simulink model "A3_2_pose"  (R2024b)
settings: Solver=ode4  StartTime=0.0  StopTime=T_run  FixedStep=Ts_ctrl  RelTol=1e-3
InitFcn:
  | if ~exist('A3_model_init','file'), addpath(fileparts(get_param('A3_2_pose','FileName'))); end, A3_model_init('A3_2_pose')
StopFcn:
  | A3_model_done('A3_2_pose')
values from neighbouring files (symbols this model uses):
  alloc_mode = 2    [A3_setup.m]
  animate = 0    [A3_setup.m]
  az_prm = [half_beam; l_thr; F_max; d_max; rev_on]    [A3_setup.m]
  beta_c = deg2rad(current_direction)    [A3_setup.m]
  current_speed = 0    [A3_setup.m]
  d_rate = deg2rad(d_rate_deg)    [A3_setup.m]
  F_max = 500    [A3_azpolar_example.m]    (also in A3_nullspace_example.m; A3_pinv_example.m; A3_setup.m)
  Kb = Ki_u/Kp_u    (= 0.333333333333)    [A3_setup.m]
  Kd_psi = 200    [A3_setup.m]
  Ki_u = 100    [A3_setup.m]
  Ki_v = 100    [A3_setup.m]
  Kp_psi = 400    [A3_setup.m]
  Kp_u = 300    [A3_setup.m]
  Kp_v = 300    [A3_setup.m]
  Kp_x = 0.4    [A3_setup.m]
  Kp_y = 0.4    [A3_setup.m]
  N_max = 2*half_beam*F_max    (= 1027.135)    [A3_setup.m]
  R_stop = 1.5    [A3_setup.m]
  stop_hold = 15    [A3_setup.m]
  stop_q = [x_d; y_d; psi_d]    [A3_setup.m]
  Ts_ctrl = 0.05    [A3_setup.m]
  u_max = 1.5    [A3_setup.m]
  U_stop = 0.05    [A3_setup.m]
  usv_p = [m_usv; Izz; Xu; Xuu; Yv; Yvv; Nr; Nrr]    [A3_setup.m]
  v_max = 0.6    [A3_setup.m]
  x0 = [0.1; 0; 0; 0; 0; psi_init]    [A3_setup.m]    (also in tidy_layout.m = min(P(:,1)))
  Y_max = F_max / T_per_Y    [A3_setup.m]
libraries: slpidlib x2
settings Model: Creator=admin  LastModifiedBy=admin

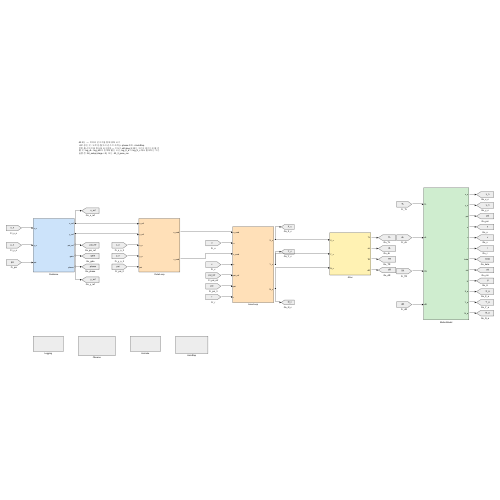
[thumbnail: Simulink's stored preview of the top-level diagram]
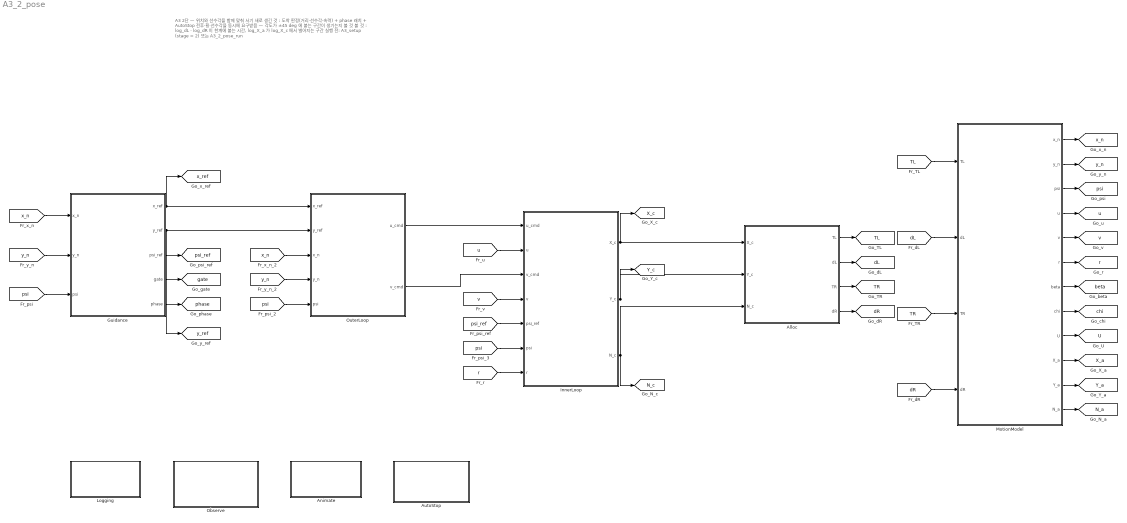
== system A3_2_pose ==
  note: A3 2단  —  위치와 선수각을 함께 맞춰 서기
      | 새로 생긴 것 : 도착 판정(거리·선수각·속력) + phase 래치 + AutoStop
      | 전후·횡·선수각을 동시에 요구받음 — 각도가 ±45 deg 에 붙는 구간이 생기는지 볼 것
      | 볼 것 : log_dL · log_dR 이 한계에 붙는 시간, log_X_a 가 log_X_c 에서 벌어지는 구간
      | 실행 전: A3_setup (stage = 2)  또는  A3_2_pose_run
  Alloc : Subsystem
  Animate : Subsystem
  AutoStop : Subsystem
  Guidance : Subsystem
  InnerLoop : Subsystem
  Logging : Subsystem
  MotionModel : Subsystem
  Observe : Subsystem
  OuterLoop : Subsystem
  tag scope: N_a=global, N_c=global, TL=global, TR=global, U=global, X_a=global, X_c=global, Y_a=global, Y_c=global, beta=global, chi=global, dL=global, dR=global, gate=global, phase=global, psi=global, psi_ref=global, r=global, u=global, v=global, x_n=global, x_ref=global, y_n=global, y_ref=global
  wires:
  InnerLoop/2(Y_c) -> Alloc/2(Y_c), [Y_c]
  OuterLoop/2(v_cmd) -> InnerLoop/3(v_cmd)
  OuterLoop/1(u_cmd) -> InnerLoop/1(u_cmd)
  Guidance/2(y_ref) -> OuterLoop/2(y_ref), [y_ref]
  Guidance/1(x_ref) -> OuterLoop/1(x_ref), [x_ref]
  InnerLoop/1(X_c) -> Alloc/1(X_c), [X_c]
  Alloc/1(TL) -> [TL]
  MotionModel/9(U) -> [U]
  MotionModel/10(X_a) -> [X_a]
  MotionModel/11(Y_a) -> [Y_a]
  MotionModel/7(beta) -> [beta]
  MotionModel/8(chi) -> [chi]
  Alloc/2(dL) -> [dL]
  Alloc/4(dR) -> [dR]
  MotionModel/3(psi) -> [psi]
  Guidance/3(psi_ref) -> [psi_ref]
  MotionModel/6(r) -> [r]
  MotionModel/4(u) -> [u]
  MotionModel/5(v) -> [v]
  MotionModel/1(x_n) -> [x_n]
  MotionModel/2(y_n) -> [y_n]
  [TL] -> MotionModel/1(TL)
  [TR] -> MotionModel/3(TR)
  [dL] -> MotionModel/2(dL)
  [dR] -> MotionModel/4(dR)
  [r] -> InnerLoop/7(r)
  [u] -> InnerLoop/2(u)
  [x_n] -> Guidance/1(x_n)
  [x_n] -> OuterLoop/3(x_n)
  [y_n] -> Guidance/2(y_n)
  [y_n] -> OuterLoop/4(y_n)
  MotionModel/12(N_a) -> [N_a]
  Alloc/3(TR) -> [TR]
  Guidance/4(gate) -> [gate]
  Guidance/5(phase) -> [phase]
  [psi] -> Guidance/3(psi)
  [psi] -> OuterLoop/5(psi)
  [psi] -> InnerLoop/6(psi)
  [psi_ref] -> InnerLoop/5(psi_ref)
  [v] -> InnerLoop/4(v)
  InnerLoop/3(N_c) -> Alloc/3(N_c), [N_c]

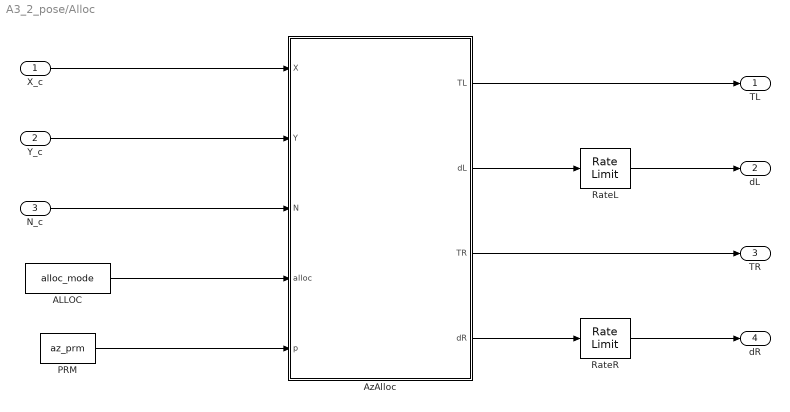
== system A3_2_pose/Alloc ==
  X_c : Inport
  Y_c : Inport  Port=2
  N_c : Inport  Port=3
  ALLOC : Constant  Value=alloc_mode
  AzAlloc : MATLAB Function  TreatAsAtomicUnit=on
  PRM : Constant  Value=az_prm
  RateL : RateLimiter  RisingSlewLimit=d_rate  FallingSlewLimit=-d_rate  SampleTimeMode=inherited
  RateR : RateLimiter  RisingSlewLimit=d_rate  FallingSlewLimit=-d_rate  SampleTimeMode=inherited
  TL : Outport
  dL : Outport  Port=2
  TR : Outport  Port=3
  dR : Outport  Port=4
  wires:
  X_c/1 -> AzAlloc/1(X)
  Y_c/1 -> AzAlloc/2(Y)
  N_c/1 -> AzAlloc/3(N)
  ALLOC/1 -> AzAlloc/4(alloc)
  PRM/1 -> AzAlloc/5(p)
  AzAlloc/2(dL) -> RateL/1
  AzAlloc/4(dR) -> RateR/1
  AzAlloc/1(TL) -> TL/1
  RateL/1 -> dL/1
  RateR/1 -> dR/1
  AzAlloc/3(TR) -> TR/1

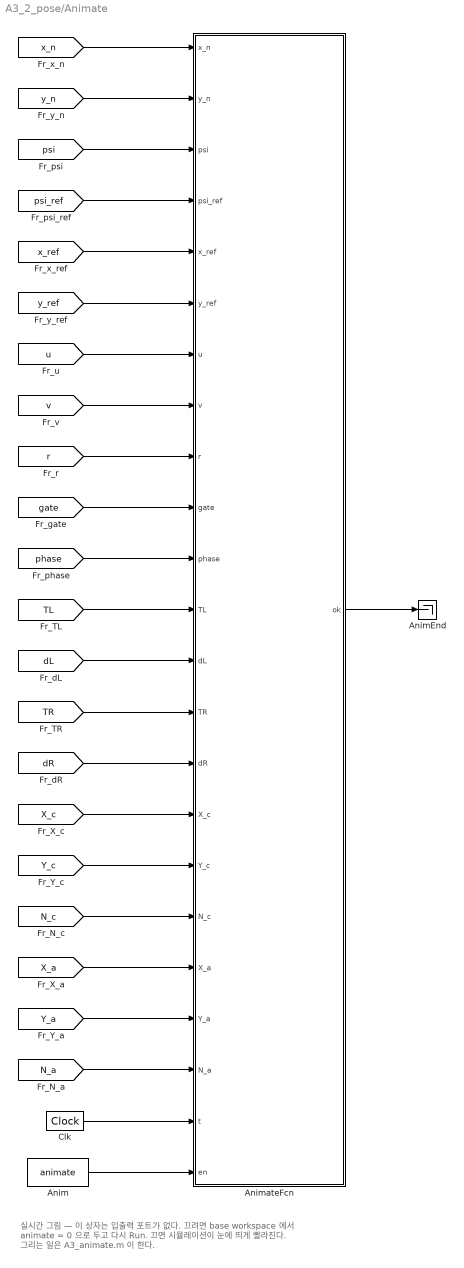
== system A3_2_pose/Animate ==
  note: 실시간 그림 — 이 상자는 입출력 포트가 없다.
      | 끄려면 base workspace 에서  animate = 0  으로 두고 다시 Run.
      | 끄면 시뮬레이션이 눈에 띄게 빨라진다.
      | 그리는 일은 A3_animate.m 이 한다.
  Anim : Constant  Value=animate
  AnimEnd : Terminator
  AnimateFcn : MATLAB Function  TreatAsAtomicUnit=on
  Clk : DigitalClock  SampleTime=Ts_ctrl
  wires:
  [x_n] -> AnimateFcn/1(x_n)
  [y_n] -> AnimateFcn/2(y_n)
  [psi] -> AnimateFcn/3(psi)
  [psi_ref] -> AnimateFcn/4(psi_ref)
  [x_ref] -> AnimateFcn/5(x_ref)
  [y_ref] -> AnimateFcn/6(y_ref)
  [u] -> AnimateFcn/7(u)
  [v] -> AnimateFcn/8(v)
  [r] -> AnimateFcn/9(r)
  [gate] -> AnimateFcn/10(gate)
  [phase] -> AnimateFcn/11(phase)
  [TL] -> AnimateFcn/12(TL)
  [dL] -> AnimateFcn/13(dL)
  [TR] -> AnimateFcn/14(TR)
  [dR] -> AnimateFcn/15(dR)
  [X_c] -> AnimateFcn/16(X_c)
  [Y_c] -> AnimateFcn/17(Y_c)
  [N_c] -> AnimateFcn/18(N_c)
  [X_a] -> AnimateFcn/19(X_a)
  [Y_a] -> AnimateFcn/20(Y_a)
  [N_a] -> AnimateFcn/21(N_a)
  Clk/1 -> AnimateFcn/22(t)
  Anim/1 -> AnimateFcn/23(en)
  AnimateFcn/1(ok) -> AnimEnd/1

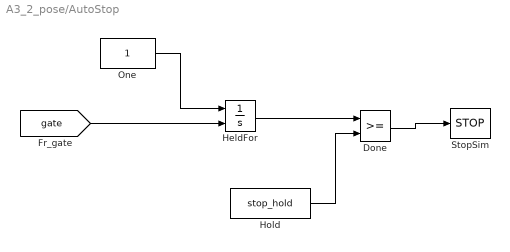
== system A3_2_pose/AutoStop ==
  Done : RelationalOperator  OutDataTypeStr=boolean  RndMeth=Simplest  InputSameDT=off
  HeldFor : Integrator  ExternalReset=level
  Hold : Constant  Value=stop_hold
  One : Constant
  StopSim : Stop
  wires:
  One/1 -> HeldFor/1
  [gate] -> HeldFor/2
  HeldFor/1 -> Done/1
  Hold/1 -> Done/2
  Done/1 -> StopSim/1

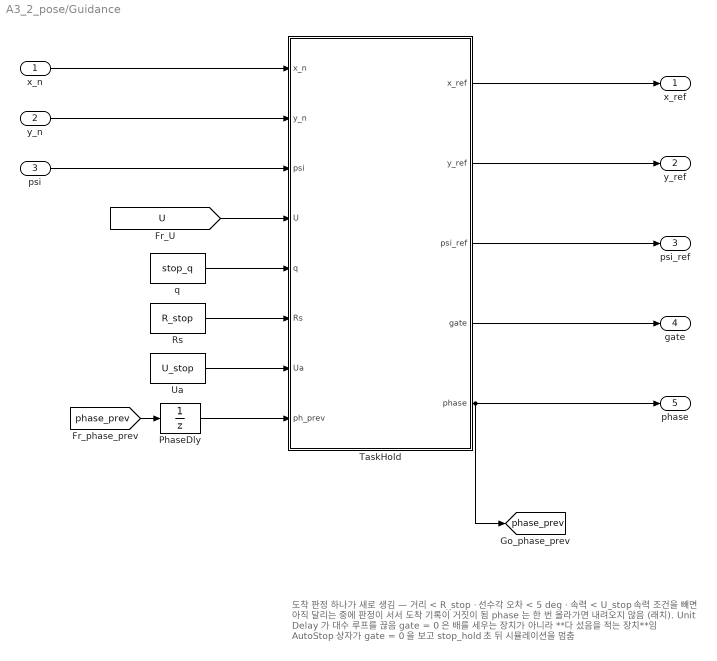
== system A3_2_pose/Guidance ==
  note: 도착 판정 하나가 새로 생김 — 거리 < R_stop · 선수각 오차 < 5 deg · 속력 < U_stop
      | 속력 조건을 빼면 아직 달리는 중에 판정이 서서 도착 기록이 거짓이 됨
      | phase 는 한 번 올라가면 내려오지 않음 (래치). Unit Delay 가 대수 루프를 끊음
      | gate = 0 은 배를 세우는 장치가 아니라 **다 섰음을 적는 장치**임
      | AutoStop 상자가 gate = 0 을 보고 stop_hold 초 뒤 시뮬레이션을 멈춤
  x_n : Inport
  y_n : Inport  Port=2
  psi : Inport  Port=3
  PhaseDly : UnitDelay  Description=phase 래치가 자기 자신을 입력으로 받으므로 그대로 되먹이면 대수 루프가 된다. 한 스텝 전 값을 쓰는 것 말고는 끊을 방법이 없는 자리다. 표본 간격을 고정 스텝(Ts_ctrl)과 같게 두어 연속 솔버(ode4)와 어긋나지 않는다.  SampleTime=Ts_ctrl  HasFrameUpgradeWarning=on
  Rs : Constant  Value=R_stop
  TaskHold : MATLAB Function  TreatAsAtomicUnit=on
  Ua : Constant  Value=U_stop
  q : Constant  Value=stop_q
  x_ref : Outport
  y_ref : Outport  Port=2
  psi_ref : Outport  Port=3
  gate : Outport  Port=4
  phase : Outport  Port=5
  tag scope: phase_prev=global
  wires:
  x_n/1 -> TaskHold/1(x_n)
  y_n/1 -> TaskHold/2(y_n)
  psi/1 -> TaskHold/3(psi)
  [U] -> TaskHold/4(U)
  q/1 -> TaskHold/5(q)
  Rs/1 -> TaskHold/6(Rs)
  Ua/1 -> TaskHold/7(Ua)
  PhaseDly/1 -> TaskHold/8(ph_prev)
  TaskHold/1(x_ref) -> x_ref/1
  TaskHold/2(y_ref) -> y_ref/1
  TaskHold/3(psi_ref) -> psi_ref/1
  TaskHold/4(gate) -> gate/1
  TaskHold/5(phase) -> phase/1, [phase_prev]
  [phase_prev] -> PhaseDly/1

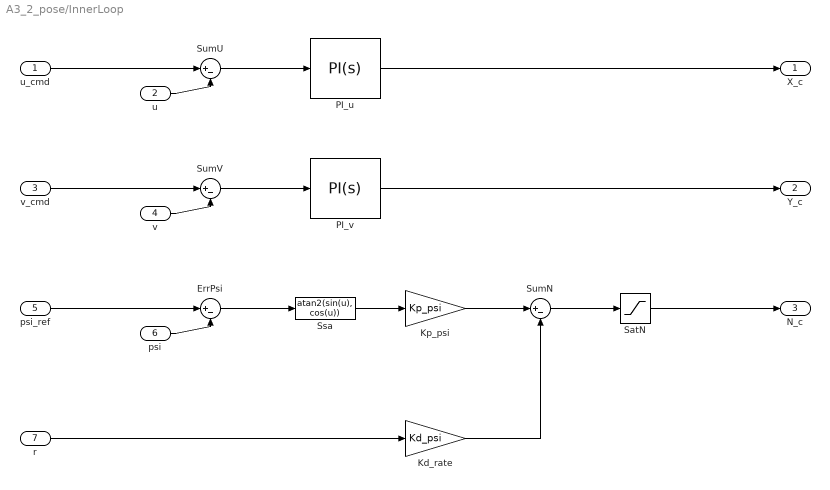
== system A3_2_pose/InnerLoop ==
  u_cmd : Inport
  u : Inport  Port=2
  v_cmd : Inport  Port=3
  v : Inport  Port=4
  psi_ref : Inport  Port=5
  psi : Inport  Port=6
  r : Inport  Port=7
  ErrPsi : Sum  Inputs=|+-
  Kd_rate : Gain  Gain=Kd_psi
  Kp_psi : Gain  Gain=Kp_psi
  PI_u : slpidlib/PID Controller  Controller=PI  Form=Parallel  TimeDomain=Continuous-time  UseExternalTs=off  SampleTime=-1  IntegratorMethod=Forward Euler  FilterMethod=Forward Euler  ControllerParametersSource=internal  P=Kp_u  I=Ki_u  UseKiTs=off  D=0  UseExternalDerivativeSource=off  N=100  UseFilter=on  TunerSelectOption=Transfer Function Based (PID Tuner App)  InitialConditionSource=internal  InitialConditionForIntegrator=0  InitialConditionForFilter=0  DifferentiatorICPrevScaledInput=0  ExternalReset=none  TrackingMode=off  Kt=1  LimitOutput=on  SatLimitsSource=internal  UpperSaturationLimit=2*F_max  LowerSaturationLimit=-(2*F_max)  LinearizeAsGain=on  AntiWindupMode=back-calculation  Kb=Kb  LimitIntegrator=off  UpperIntegratorSaturationLimit=inf  LowerIntegratorSaturationLimit=-inf  POutMin=[]  POutMax=[]  IOutMin=[]  IOutMax=[]  DOutMin=[]  DOutMax=[]  NOutMin=[]  NOutMax=[]  SumOutMin=[]  SumOutMax=[]  SaturationOutMin=[]  SaturationOutMax=[]  PParamMin=[]  PParamMax=[]  IParamMin=[]  IParamMax=[]  DParamMin=[]  DParamMax=[]  NParamMin=[]  NParamMax=[]  KbParamMin=[]  KbParamMax=[]  KtParamMin=[]  KtParamMax=[]  KbOutMin=[]  KbOutMax=[]  KtOutMin=[]  KtOutMax=[]  IntegratorOutMin=[]  IntegratorOutMax=[]  FilterOutMin=[]  FilterOutMax=[]  SumI1OutMin=[]  SumI1OutMax=[]  SumI2OutMin=[]  SumI2OutMax=[]  SumI3OutMin=[]  SumI3OutMax=[]  SumI4OutMin=[]  SumI4OutMax=[]  SumDOutMin=[]  SumDOutMax=[]  DifferentiatorOutMin=[]  DifferentiatorOutMax=[]  FilterDiffOutCoefMin=[]  FilterDiffOutCoefMax=[]  ReciprocalOutMin=[]  ReciprocalOutMax=[]  SumDenOutMin=[]  SumDenOutMax=[]  SumNumOutMin=[]  SumNumOutMax=[]  DivideOutMin=[]  DivideOutMax=[]  UdiffTsProdOutMin=[]  UdiffTsProdOutMax=[]  NTsProdOutMin=[]  NTsProdOutMax=[]  UintegralTsProdOutMin=[]  UintegralTsProdOutMax=[]  UngainTsProdOutMin=[]  UngainTsProdOutMax=[]  ClampingZeroOutDataTypeStr=Inherit: Inherit via back propagation  ClampingZeroOutMin=[]  ClampingZeroOutMax=[]  FilterDenConstantOutDataTypeStr=Inherit: Inherit via back propagation  FilterDenConstantOutMin=[]  FilterDenConstantOutMax=[]  PCopyOutDataTypeStr=Inherit: Inherit via back propagation  PCopyOutMin=[]  PCopyOutMax=[]  NCopyOutDataTypeStr=Inherit: Inherit via back propagation  NCopyOutMin=[]  NCopyOutMax=[]  IntegratorContinuousStateAttributes=''  IntegratorStateMustResolveToSignalObject=off  IntegratorRTWStateStorageClass=Auto  FilterContinuousStateAttributes=''  FilterStateMustResolveToSignalObject=off  FilterRTWStateStorageClass=Auto  ParallelPVariant=InternalParameters  IdealPVariant=Disabled  IVariant=InternalParameters  DVariant=Disabled  IntegratorVariant=Continuous  SatVariant=Enabled  AWVariant=BackCalculation  PCopyVariant=Disabled  TRVariant=Disabled  FdbkBlocksVariant=Forward  IdealPFdbkVariant=Disabled  SatFdbkVariant=Disabled  DerivativeFilterVariant=Disabled  NVariant=Disabled  NCopyVariant=Disabled_SignalSpec  FilterICVariant=Disabled  IntegratorICVariant=InternalICs  ExternalResetVariant=Disabled  TRSumVariant=Passthrough  SumFdbkVariant=Disabled  SumVariant=Sum_PI  TsampFilterVariant=InternalTs  TsampNgainVariant=Passthrough  TsampIntegralVariant=Disabled_SignalSpec  ExternalSaturationOutDataTypeStr=Inherit: Same as second input  DerivativeSourceVariant=Disabled  PreIntVariant=InternalPreInt
  PI_v : slpidlib/PID Controller  Controller=PI  Form=Parallel  TimeDomain=Continuous-time  UseExternalTs=off  SampleTime=-1  IntegratorMethod=Forward Euler  FilterMethod=Forward Euler  ControllerParametersSource=internal  P=Kp_v  I=Ki_v  UseKiTs=off  D=0  UseExternalDerivativeSource=off  N=100  UseFilter=on  TunerSelectOption=Transfer Function Based (PID Tuner App)  InitialConditionSource=internal  InitialConditionForIntegrator=0  InitialConditionForFilter=0  DifferentiatorICPrevScaledInput=0  ExternalReset=none  TrackingMode=off  Kt=1  LimitOutput=on  SatLimitsSource=internal  UpperSaturationLimit=Y_max  LowerSaturationLimit=-(Y_max)  LinearizeAsGain=on  AntiWindupMode=back-calculation  Kb=Kb  LimitIntegrator=off  UpperIntegratorSaturationLimit=inf  LowerIntegratorSaturationLimit=-inf  POutMin=[]  POutMax=[]  IOutMin=[]  IOutMax=[]  DOutMin=[]  DOutMax=[]  NOutMin=[]  NOutMax=[]  SumOutMin=[]  SumOutMax=[]  SaturationOutMin=[]  SaturationOutMax=[]  PParamMin=[]  PParamMax=[]  IParamMin=[]  IParamMax=[]  DParamMin=[]  DParamMax=[]  NParamMin=[]  NParamMax=[]  KbParamMin=[]  KbParamMax=[]  KtParamMin=[]  KtParamMax=[]  KbOutMin=[]  KbOutMax=[]  KtOutMin=[]  KtOutMax=[]  IntegratorOutMin=[]  IntegratorOutMax=[]  FilterOutMin=[]  FilterOutMax=[]  SumI1OutMin=[]  SumI1OutMax=[]  SumI2OutMin=[]  SumI2OutMax=[]  SumI3OutMin=[]  SumI3OutMax=[]  SumI4OutMin=[]  SumI4OutMax=[]  SumDOutMin=[]  SumDOutMax=[]  DifferentiatorOutMin=[]  DifferentiatorOutMax=[]  FilterDiffOutCoefMin=[]  FilterDiffOutCoefMax=[]  ReciprocalOutMin=[]  ReciprocalOutMax=[]  SumDenOutMin=[]  SumDenOutMax=[]  SumNumOutMin=[]  SumNumOutMax=[]  DivideOutMin=[]  DivideOutMax=[]  UdiffTsProdOutMin=[]  UdiffTsProdOutMax=[]  NTsProdOutMin=[]  NTsProdOutMax=[]  UintegralTsProdOutMin=[]  UintegralTsProdOutMax=[]  UngainTsProdOutMin=[]  UngainTsProdOutMax=[]  ClampingZeroOutDataTypeStr=Inherit: Inherit via back propagation  ClampingZeroOutMin=[]  ClampingZeroOutMax=[]  FilterDenConstantOutDataTypeStr=Inherit: Inherit via back propagation  FilterDenConstantOutMin=[]  FilterDenConstantOutMax=[]  PCopyOutDataTypeStr=Inherit: Inherit via back propagation  PCopyOutMin=[]  PCopyOutMax=[]  NCopyOutDataTypeStr=Inherit: Inherit via back propagation  NCopyOutMin=[]  NCopyOutMax=[]  IntegratorContinuousStateAttributes=''  IntegratorStateMustResolveToSignalObject=off  IntegratorRTWStateStorageClass=Auto  FilterContinuousStateAttributes=''  FilterStateMustResolveToSignalObject=off  FilterRTWStateStorageClass=Auto  ParallelPVariant=InternalParameters  IdealPVariant=Disabled  IVariant=InternalParameters  DVariant=Disabled  IntegratorVariant=Continuous  SatVariant=Enabled  AWVariant=BackCalculation  PCopyVariant=Disabled  TRVariant=Disabled  FdbkBlocksVariant=Forward  IdealPFdbkVariant=Disabled  SatFdbkVariant=Disabled  DerivativeFilterVariant=Disabled  NVariant=Disabled  NCopyVariant=Disabled_SignalSpec  FilterICVariant=Disabled  IntegratorICVariant=InternalICs  ExternalResetVariant=Disabled  TRSumVariant=Passthrough  SumFdbkVariant=Disabled  SumVariant=Sum_PI  TsampFilterVariant=InternalTs  TsampNgainVariant=Passthrough  TsampIntegralVariant=Disabled_SignalSpec  ExternalSaturationOutDataTypeStr=Inherit: Same as second input  DerivativeSourceVariant=Disabled  PreIntVariant=InternalPreInt
  SatN : Saturate  UpperLimit=N_max  LowerLimit=-(N_max)
  Ssa : Fcn  Expr=atan2(sin(u), cos(u))
  SumN : Sum  Inputs=|+-
  SumU : Sum  Inputs=|+-
  SumV : Sum  Inputs=|+-
  X_c : Outport
  Y_c : Outport  Port=2
  N_c : Outport  Port=3
  wires:
  u_cmd/1 -> SumU/1
  u/1 -> SumU/2
  v_cmd/1 -> SumV/1
  v/1 -> SumV/2
  SumU/1 -> PI_u/1
  SumV/1 -> PI_v/1
  ErrPsi/1 -> Ssa/1
  psi_ref/1 -> ErrPsi/1
  psi/1 -> ErrPsi/2
  Ssa/1 -> Kp_psi/1
  r/1 -> Kd_rate/1
  Kp_psi/1 -> SumN/1
  Kd_rate/1 -> SumN/2
  SumN/1 -> SatN/1
  PI_u/1 -> X_c/1
  SatN/1 -> N_c/1
  PI_v/1 -> Y_c/1

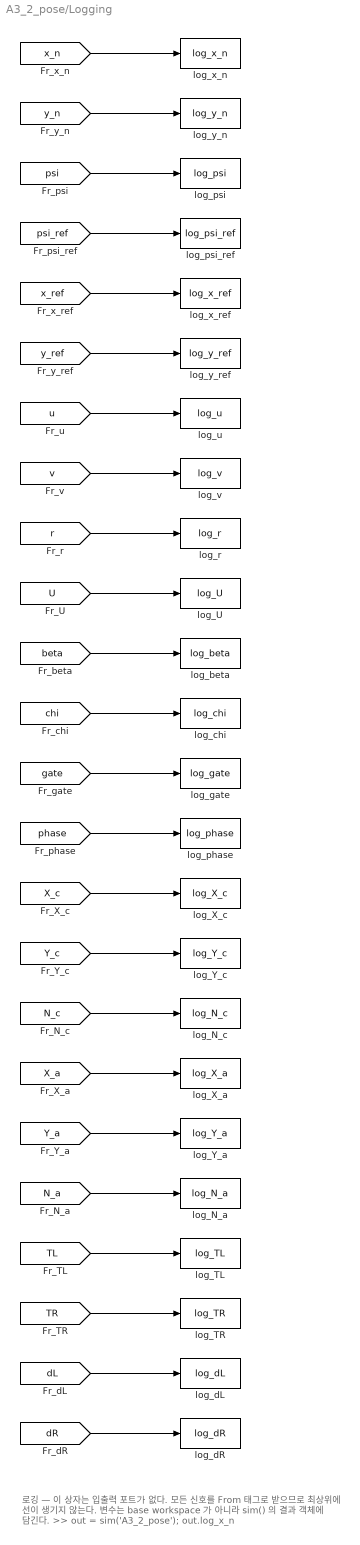
== system A3_2_pose/Logging ==
  note: 로깅 — 이 상자는 입출력 포트가 없다.
      | 모든 신호를 From 태그로 받으므로 최상위에 선이 생기지 않는다.
      | 변수는 base workspace 가 아니라 sim() 의 결과 객체에 담긴다.
      |   >> out = sim('A3_2_pose');  out.log_x_n
  log_N_a : ToWorkspace  VariableName=log_N_a  SaveFormat=Timeseries  SampleTime=Ts_ctrl
  log_N_c : ToWorkspace  VariableName=log_N_c  SaveFormat=Timeseries  SampleTime=Ts_ctrl
  log_TL : ToWorkspace  VariableName=log_TL  SaveFormat=Timeseries  SampleTime=Ts_ctrl
  log_TR : ToWorkspace  VariableName=log_TR  SaveFormat=Timeseries  SampleTime=Ts_ctrl
  log_U : ToWorkspace  VariableName=log_U  SaveFormat=Timeseries  SampleTime=Ts_ctrl
  log_X_a : ToWorkspace  VariableName=log_X_a  SaveFormat=Timeseries  SampleTime=Ts_ctrl
  log_X_c : ToWorkspace  VariableName=log_X_c  SaveFormat=Timeseries  SampleTime=Ts_ctrl
  log_Y_a : ToWorkspace  VariableName=log_Y_a  SaveFormat=Timeseries  SampleTime=Ts_ctrl
  log_Y_c : ToWorkspace  VariableName=log_Y_c  SaveFormat=Timeseries  SampleTime=Ts_ctrl
  log_beta : ToWorkspace  VariableName=log_beta  SaveFormat=Timeseries  SampleTime=Ts_ctrl
  log_chi : ToWorkspace  VariableName=log_chi  SaveFormat=Timeseries  SampleTime=Ts_ctrl
  log_dL : ToWorkspace  VariableName=log_dL  SaveFormat=Timeseries  SampleTime=Ts_ctrl
  log_dR : ToWorkspace  VariableName=log_dR  SaveFormat=Timeseries  SampleTime=Ts_ctrl
  log_gate : ToWorkspace  VariableName=log_gate  SaveFormat=Timeseries  SampleTime=Ts_ctrl
  log_phase : ToWorkspace  VariableName=log_phase  SaveFormat=Timeseries  SampleTime=Ts_ctrl
  log_psi : ToWorkspace  VariableName=log_psi  SaveFormat=Timeseries  SampleTime=Ts_ctrl
  log_psi_ref : ToWorkspace  VariableName=log_psi_ref  SaveFormat=Timeseries  SampleTime=Ts_ctrl
  log_r : ToWorkspace  VariableName=log_r  SaveFormat=Timeseries  SampleTime=Ts_ctrl
  log_u : ToWorkspace  VariableName=log_u  SaveFormat=Timeseries  SampleTime=Ts_ctrl
  log_v : ToWorkspace  VariableName=log_v  SaveFormat=Timeseries  SampleTime=Ts_ctrl
  log_x_n : ToWorkspace  VariableName=log_x_n  SaveFormat=Timeseries  SampleTime=Ts_ctrl
  log_x_ref : ToWorkspace  VariableName=log_x_ref  SaveFormat=Timeseries  SampleTime=Ts_ctrl
  log_y_n : ToWorkspace  VariableName=log_y_n  SaveFormat=Timeseries  SampleTime=Ts_ctrl
  log_y_ref : ToWorkspace  VariableName=log_y_ref  SaveFormat=Timeseries  SampleTime=Ts_ctrl
  wires:
  [x_n] -> log_x_n/1
  [y_n] -> log_y_n/1
  [psi] -> log_psi/1
  [psi_ref] -> log_psi_ref/1
  [x_ref] -> log_x_ref/1
  [y_ref] -> log_y_ref/1
  [u] -> log_u/1
  [v] -> log_v/1
  [r] -> log_r/1
  [U] -> log_U/1
  [beta] -> log_beta/1
  [chi] -> log_chi/1
  [gate] -> log_gate/1
  [phase] -> log_phase/1
  [X_c] -> log_X_c/1
  [Y_c] -> log_Y_c/1
  [N_c] -> log_N_c/1
  [X_a] -> log_X_a/1
  [Y_a] -> log_Y_a/1
  [N_a] -> log_N_a/1
  [TL] -> log_TL/1
  [TR] -> log_TR/1
  [dL] -> log_dL/1
  [dR] -> log_dR/1

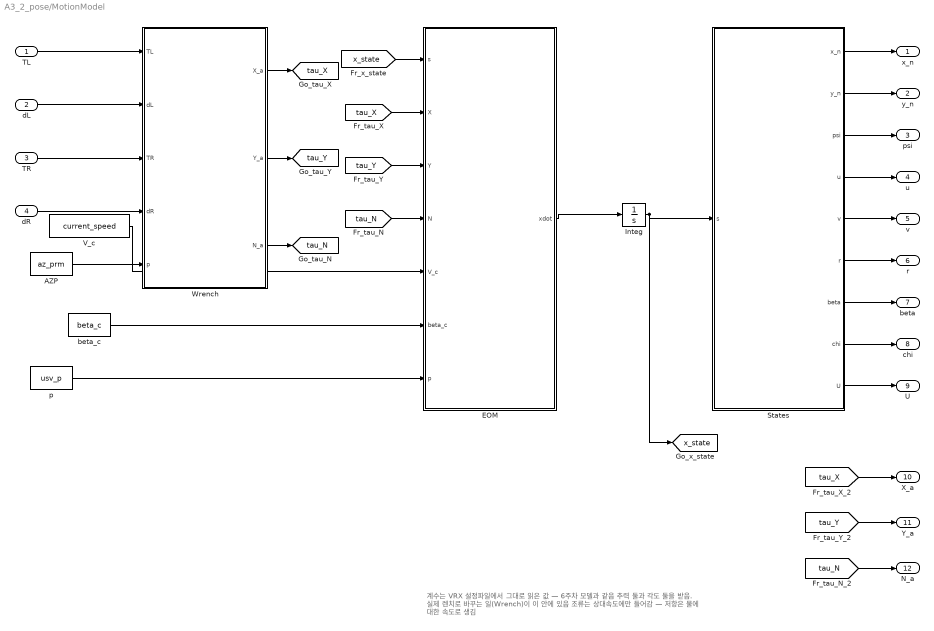
== system A3_2_pose/MotionModel ==
  note: 계수는 VRX 설정파일에서 그대로 읽은 값 — 6주차 모델과 같음
      | 추력 둘과 각도 둘을 받음. 실제 렌치로 바꾸는 일(Wrench)이 이 안에 있음
      | 조류는 상대속도에만 들어감 — 저항은 물에 대한 속도로 생김
  TL : Inport
  dL : Inport  Port=2
  TR : Inport  Port=3
  dR : Inport  Port=4
  AZP : Constant  Value=az_prm
  EOM : MATLAB Function  TreatAsAtomicUnit=on
  Integ : Integrator  InitialCondition=x0
  States : MATLAB Function  TreatAsAtomicUnit=on
  V_c : Constant  Value=current_speed
  Wrench : MATLAB Function  TreatAsAtomicUnit=on
  beta_c : Constant  Value=beta_c
  p : Constant  Value=usv_p
  x_n : Outport
  y_n : Outport  Port=2
  psi : Outport  Port=3
  u : Outport  Port=4
  v : Outport  Port=5
  r : Outport  Port=6
  beta : Outport  Port=7
  chi : Outport  Port=8
  U : Outport  Port=9
  X_a : Outport  Port=10
  Y_a : Outport  Port=11
  N_a : Outport  Port=12
  tag scope: tau_N=global, tau_X=global, tau_Y=global, x_state=global
  wires:
  TL/1 -> Wrench/1(TL)
  dL/1 -> Wrench/2(dL)
  TR/1 -> Wrench/3(TR)
  dR/1 -> Wrench/4(dR)
  AZP/1 -> Wrench/5(p)
  Wrench/1(X_a) -> [tau_X]
  Wrench/2(Y_a) -> [tau_Y]
  Wrench/3(N_a) -> [tau_N]
  [tau_X] -> EOM/2(X)
  [tau_Y] -> EOM/3(Y)
  [tau_N] -> EOM/4(N)
  V_c/1 -> EOM/5(V_c)
  beta_c/1 -> EOM/6(beta_c)
  p/1 -> EOM/7(p)
  EOM/1(xdot) -> Integ/1
  Integ/1 -> States/1(s), [x_state]
  [x_state] -> EOM/1(s)
  States/1(x_n) -> x_n/1
  States/2(y_n) -> y_n/1
  States/3(psi) -> psi/1
  States/4(u) -> u/1
  States/5(v) -> v/1
  States/6(r) -> r/1
  States/7(beta) -> beta/1
  States/8(chi) -> chi/1
  States/9(U) -> U/1
  [tau_X] -> X_a/1
  [tau_Y] -> Y_a/1
  [tau_N] -> N_a/1

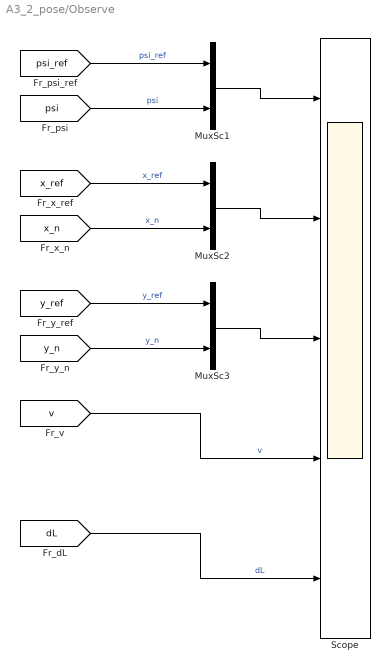
== system A3_2_pose/Observe ==
  MuxSc1 : Mux  Inputs=2
  MuxSc2 : Mux  Inputs=2
  MuxSc3 : Mux  Inputs=2
  Scope : Scope  NumInputPorts=5
  wires:
  [psi_ref] -> MuxSc1/1  "psi_ref"
  [psi] -> MuxSc1/2  "psi"
  MuxSc1/1 -> Scope/1
  [x_ref] -> MuxSc2/1  "x_ref"
  [x_n] -> MuxSc2/2  "x_n"
  MuxSc2/1 -> Scope/2
  [y_ref] -> MuxSc3/1  "y_ref"
  [y_n] -> MuxSc3/2  "y_n"
  MuxSc3/1 -> Scope/3
  [v] -> Scope/4  "v"
  [dL] -> Scope/5  "dL"

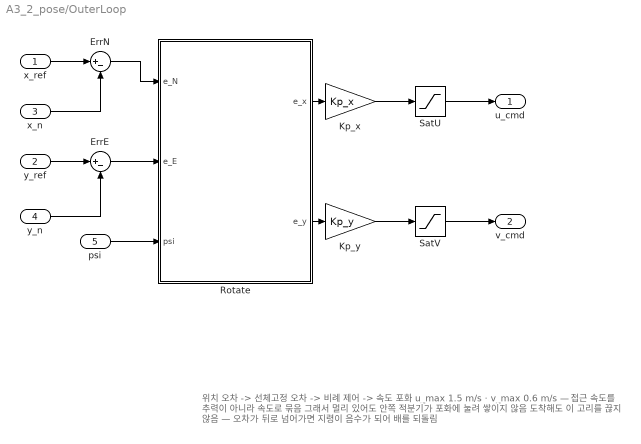
== system A3_2_pose/OuterLoop ==
  note: 위치 오차 -> 선체고정 오차 -> 비례 제어 -> 속도 포화
      | u_max 1.5 m/s · v_max 0.6 m/s — 접근 속도를 추력이 아니라 속도로 묶음
      | 그래서 멀리 있어도 안쪽 적분기가 포화에 눌려 쌓이지 않음
      | 도착해도 이 고리를 끊지 않음 — 오차가 뒤로 넘어가면 지령이 음수가 되어 배를 되돌림
  x_ref : Inport
  y_ref : Inport  Port=2
  x_n : Inport  Port=3
  y_n : Inport  Port=4
  psi : Inport  Port=5
  ErrE : Sum  Inputs=|+-
  ErrN : Sum  Inputs=|+-
  Kp_x : Gain  Gain=Kp_x
  Kp_y : Gain  Gain=Kp_y
  Rotate : MATLAB Function  TreatAsAtomicUnit=on
  SatU : Saturate  UpperLimit=u_max  LowerLimit=-(u_max)
  SatV : Saturate  UpperLimit=v_max  LowerLimit=-(v_max)
  u_cmd : Outport
  v_cmd : Outport  Port=2
  wires:
  x_ref/1 -> ErrN/1
  Rotate/1(e_x) -> Kp_x/1
  Rotate/2(e_y) -> Kp_y/1
  ErrE/1 -> Rotate/2(e_E)
  x_n/1 -> ErrN/2
  y_ref/1 -> ErrE/1
  ErrN/1 -> Rotate/1(e_N)
  y_n/1 -> ErrE/2
  psi/1 -> Rotate/3(psi)
  Kp_x/1 -> SatU/1
  Kp_y/1 -> SatV/1
  SatU/1 -> u_cmd/1
  SatV/1 -> v_cmd/1

== matlab function A3_2_pose/Animate/AnimateFcn ==
  data: x_n input; y_n input; psi input; psi_ref input; x_ref input; y_ref input; u input; ok output; v input; r input; gate input; phase input; TL input; dL input; TR input; dR input; X_c input; Y_c input; N_c input; X_a input; Y_a input; N_a input; t input; en input
function ok = AnimateFcn(x_n, y_n, psi, psi_ref, x_ref, y_ref, u, v, r, gate, phase, TL, dL, TR, dR, X_c, Y_c, N_c, X_a, Y_a, N_a, t, en)
%#codegen
% Live plot while the model runs. A MATLAB Function block cannot
% plot, so the drawing function is declared extrinsic: Simulink
% calls plain MATLAB instead of generating code for it.
coder.extrinsic('A3_animate');
ok = 1;
if en > 0.5
    A3_animate(x_n, y_n, psi, psi_ref, x_ref, y_ref, u, v, r, gate, phase, TL, dL, TR, dR, X_c, Y_c, N_c, X_a, Y_a, N_a, t);
end

== matlab function A3_2_pose/OuterLoop/Rotate ==
  data: e_N input; e_x output; e_E input; psi input; e_y output
function [e_x, e_y] = Rotate(e_N, e_E, psi)
%#codegen
%  NED 위치 오차를 선체고정 오차로 돌린다. e_x 앞쪽, e_y 우현쪽 [m]
e_x =  cos(psi)*e_N + sin(psi)*e_E;
e_y = -sin(psi)*e_N + cos(psi)*e_E;

== matlab function A3_2_pose/Guidance/TaskHold ==
  data: x_n input; x_ref output; y_n input; psi input; U input; q input; Rs input; Ua input; ph_prev input; y_ref output; psi_ref output; gate output; phase output
function [x_ref, y_ref, psi_ref, gate, phase] = TaskHold(x_n, y_n, psi, U, q, Rs, Ua, ph_prev)
%#codegen
%  한 점·한 선수각을 목표로 주고, 거기 가서 **섰는지** 판정한다.
%
%    U  = 대지속력 [m/s]      운동모델이 낸 sqrt(u^2 + v^2)
%    q  = [x_d; y_d; psi_d]   목표 자세 (psi_d 는 rad)
%    Rs = R_stop              도착으로 보는 반지름 [m]
%    Ua = U_stop              도착으로 보는 속력 한계 [m/s]
%
%  gate = 1 이면 바깥 고리가 속도 지령을 낸다. 0 이면 0 을 내어 배가 선다.
x_ref = q(1);  y_ref = q(2);  psi_ref = q(3);
d = sqrt((x_ref - x_n)^2 + (y_ref - y_n)^2);
e = atan2(sin(psi_ref - psi), cos(psi_ref - psi));
ph = ph_prev;
if ph < 1 && d < Rs && abs(e) < 5*pi/180 && U < Ua
    ph = 1;                   %  도착 — 한 번 올라가면 내려오지 않는다
end
phase = ph;
gate  = double(ph < 1);

== matlab function A3_2_pose/Alloc/AzAlloc ==
  data: X input; TL output; Y input; N input; alloc input; p input; dL output; TR output; dR output
function [TL, dL, TR, dR] = AzAlloc(X, Y, N, alloc, p)
%#codegen
%  아지무스 추진기 둘에 요구 렌치를 나누어 준다
%
%  == 입력 ==============================================================
%    X      요구 전후 힘   [N]      선수 방향(+앞)
%    Y      요구 횡 힘     [N]      우현 방향(+오른쪽)
%    N      요구 요 모멘트 [N m]    시계 방향(+우선회)
%    alloc  배분 방식 [-]           1 = pseudo-inverse
%                                   2 = pseudo-inverse + null space 보정
%    p      기하·한계 묶음 (A3_setup.m 의 az_prm)
%      p(1) = b     반폭        [m]    중심선에서 추진기까지
%      p(2) = L     거리        [m]    무게중심에서 추진기까지 (뒤쪽)
%      p(3) = Fmax  추력 한계   [N]    한 대 기준
%      p(4) = dmax  각도 한계   [rad]
%      p(5) = rev   추력 반전   [-]    1 = 허용, 0 = 금지
%
%  == 출력 ==============================================================
%    TL, TR   좌·우 추력   [N]    양수면 노즐이 보는 쪽으로 민다
%    dL, dR   좌·우 각도   [rad]  선수 기준, 우현 쪽이 +
%
%  == 왜 추력과 각도를 바로 풀지 않는가 ================================
%    추진기 한 대의 힘은 극좌표 (T, d) 로 쓰면 비선형이다
%        Fx = T cos(d),   Fy = T sin(d)
%    그래서 추력과 각도를 묶어 **직교 성분 넷**을 미지수로 둔다
%        ue = [Fx_L; Fy_L; Fx_R; Fy_R]        (확장 추력 벡터)
%    이렇게 두면 요구 렌치와의 관계가 **완전한 선형식**이 된다
%        B ue = tau,   tau = [X; Y; N]
%    B 의 각 열은 "그 성분 1 N 이 렌치에 얼마를 보태는가" 이다
%    풀고 난 뒤에 극좌표로 되돌리면 추력과 각도가 나온다 (3 단계)
%    이 방식은 Sarda 등 [1] 6 절이 실제 WAM-V 에 쓴 것과 같다
%
%  == 해가 하나가 아니다 ================================================
%    미지수 4 개, 식 3 개 — 같은 렌치를 내는 해가 **직선 하나**를 이룬다
%      alloc = 1   그 직선에서 원점에 가장 가까운 점 (pseudo-inverse)
%      alloc = 2   각도 한계를 지키는 점으로 직선 위를 미끄러진다
%    직선의 방향 n = [0; 1; 0; -1] 은 좌우 횡력만 주고받는 꼴이라
%    얼마를 더해도 X, Y, N 이 한 톨도 변하지 않는다 (B n = 0)
%
%  == 참고 문헌 ==========================================================
%    [1] Sarda, Qu, Bertaska, von Ellenrieder (2016)
%        "Station keeping control of an unmanned surface vehicle exposed
%         to current and wind disturbances", Ocean Engineering 127, 305-324
%        6 절 — 아지무스 WAM-V 의 확장 추력 벡터와 pseudo-inverse 배분
%    [2] Sordalen (1997) "Optimal thrust allocation for marine vessels",
%        Control Engineering Practice 5(9), 1223-1231 — null space 이용
%    [3] Fossen (2021) "Handbook of Marine Craft Hydrodynamics and Motion
%        Control", 2nd ed., 11 장 — 배분 행렬과 pseudo-inverse 일반론

b = p(1);  L = p(2);  Fmax = p(3);  dmax = p(4);  rev = p(5);

tau = [X; Y; N];

%  배분 행렬 — 열 하나가 성분 하나의 몫이다
%    1 행 전후 · 2 행 횡 · 3 행 요 모멘트
%    좌현은 (x, y) = (-L, -b), 우현은 (-L, +b) 에 앉는다
B = [ 1,  0,  1,  0; ...
      0,  1,  0,  1; ...
      b, -L, -b, -L];

%  === 1 단계. pseudo-inverse — 크기가 가장 작은 해 ===================
%    ue = B' (B B')^-1 tau.  해의 직선에서 원점에 가장 가까운 점이다
ue = B' * ((B*B') \ tau);

%  === 2 단계. null space 보정 (alloc = 2) ============================
%    각도 한계는 |Fy| <= tan(dmax) |Fx| 와 같은 말이다.
%    ue + lam*n 을 넣으면 lam 에 대해 1 차식이라 허용 구간이 바로 나온다
if alloc > 1.5
    nz = [0; 1; 0; -1];
    td = tan(dmax);
    lo = max(-td*abs(ue(1)) - ue(2),  ue(4) - td*abs(ue(3)));
    hi = min( td*abs(ue(1)) - ue(2),  ue(4) + td*abs(ue(3)));
    if lo <= hi
        lam = min(max(0, lo), hi);     % 구간 안에서 0 에 가장 가까운 값
    else
        lam = (lo + hi)/2;             % 구간이 비면 가운데 — 덜 넘긴다
    end
    ue = ue + lam*nz;
end

%  === 3 단계. 극좌표로 되돌리고 한계 안으로 넣는다 ===================
[TL, dL] = az_polar(ue(1), ue(2), Fmax, dmax, rev);
[TR, dR] = az_polar(ue(3), ue(4), Fmax, dmax, rev);


function [T, d] = az_polar(Fx, Fy, Fmax, dmax, rev)
%  직교 성분 둘 -> 추력 하나와 각도 하나
T = hypot(Fx, Fy);
d = atan2(Fy, Fx);

%  뒤쪽을 보라는 요구는 **앞을 보고 역추력** 으로 바꿔 쓴다 (같은 힘)
if abs(d) > pi/2
    d = d - sign(d)*pi;
    T = -T;
end

%  역추력을 금지했으면 되돌린다 — 각도가 한계를 넘게 된다 (A3-4 실습)
if rev < 0.5 && T < 0
    T = -T;
    d = d + sign(d + (d==0))*pi;
    if d >  pi, d = d - 2*pi; end
    if d < -pi, d = d + 2*pi; end
end

%  한계 — 각도와 추력을 각각 한 줄로 깎는다
%    깎인 만큼이 "못 낸 힘" 으로 남아 운동모델 쪽 기록에 숫자로 보인다
d = max(min(d,  dmax), -dmax);
T = max(min(T,  Fmax), -Fmax);

== matlab function A3_2_pose/MotionModel/Wrench ==
  data: TL input; X_a output; dL input; TR input; dR input; p input; Y_a output; N_a output
function [X_a, Y_a, N_a] = Wrench(TL, dL, TR, dR, p)
%#codegen
%  추진기 명령 -> 선체에 걸리는 렌치 (운동모델의 입구)
%
%  == 입력 ==============================================================
%    TL, TR   좌·우 추력 [N]      배분기가 낸 값. 음수면 역추력
%    dL, dR   좌·우 각도 [rad]    변화율 제한을 거친 실제 각도
%    p        기하 묶음 — p(1) = b 반폭 [m], p(2) = L 거리 [m]
%
%  == 출력 ==============================================================
%    X_a  실제 전후 힘   [N]
%    Y_a  실제 횡 힘     [N]
%    N_a  실제 요 모멘트 [N m]
%
%  == 왜 운동모델 안에 있는가 ===========================================
%    선체가 받는 것은 추력과 각도가 아니라 **힘과 모멘트**다. 추진기가
%    어떻게 달려 있는지가 그 변환을 정하므로, 변환은 배(운동모델) 쪽에
%    속한다. 배분기는 "무엇을 명령할까" 까지만 책임진다
%
%  == 배분기와 같은 행렬이다 ============================================
%    배분기는 B ue = tau 를 **거꾸로** 풀었고, 여기서는 **바로** 쓴다
%        ue = [TL cos(dL); TL sin(dL); TR cos(dR); TR sin(dR)]
%        tau_a = B ue
%    각도·추력 한계에 물리지 않으면 tau_a 가 요구 렌치와 같아진다.
%    기하를 고칠 때는 azAllocFcn.m 의 B 와 **함께** 고쳐야 한다

b = p(1);  L = p(2);

B = [ 1,  0,  1,  0; ...
      0,  1,  0,  1; ...
      b, -L, -b, -L];

%  극좌표(추력·각도) -> 직교 성분 넷
ue = [TL*cos(dL); TL*sin(dL); TR*cos(dR); TR*sin(dR)];

tau_a = B*ue;

X_a = tau_a(1);  Y_a = tau_a(2);  N_a = tau_a(3);

== matlab function A3_2_pose/MotionModel/EOM ==
  data: s input; xdot output; X input; Y input; N input; V_c input; beta_c input; p input
function xdot = EOM(s, X, Y, N, V_c, beta_c, p)
%#codegen
%  3자유도 운동방정식.  s = [u v r x_n y_n psi] 의 열벡터
%
%    X, Y, N 은 Wrench 가 낸 **실제** 렌치다 (요구가 아니다)
%    조류는 상대속도에만 들어간다 — 저항은 물에 대한 속도로 생긴다
%    부가질량은 0 으로 둔다 (VRX 설정도 0 이다)
u = s(1);  v = s(2);  r = s(3);  psi = s(6);
m_s  = p(1);  Izz = p(2);
Xu   = p(3);  Xuu = p(4);
Yv   = p(5);  Yvv = p(6);
Nr   = p(7);  Nrr = p(8);

%  조류를 선체좌표로 — 물에 대한 상대속도 u_r, v_r
u_c = V_c*cos(beta_c - psi);
v_c = V_c*sin(beta_c - psi);
u_r = u - u_c;
v_r = v - v_c;

%  저항 — 선형 + 제곱 (제곱항이 있어 속도가 커질수록 빨리 늘어난다)
Dx = (Xu + Xuu*abs(u_r))*u_r;
Dy = (Yv + Yvv*abs(v_r))*v_r;
Dn = (Nr + Nrr*abs(r))*r;

%  v*r, -u*r 은 좌표계가 함께 돌기 때문에 생기는 항이다
du = (X - Dx)/m_s + v*r;
dv = (Y - Dy)/m_s - u*r;
dr = (N - Dn)/Izz;

%  선체속도를 NED 로 — 이것이 위치의 미분이다
xdot = [du; dv; dr; ...
        u*cos(psi) - v*sin(psi); ...
        u*sin(psi) + v*cos(psi); ...
        r];

== matlab function A3_2_pose/MotionModel/States ==
  data: s input; x_n output; y_n output; psi output; u output; v output; r output; beta output; chi output; U output
function [x_n, y_n, psi, u, v, r, beta, chi, U] = States(s)
%#codegen
%  상태벡터를 쓰기 좋은 이름으로 풀어 놓는다.
%    U    대지속력 [m/s]
%    beta 크랩각 — 뱃머리와 실제 가는 방향의 차이 [rad]
%    chi  침로 = psi + beta, 실제 가는 방향 [rad]
%  순수 횡이동에서는 beta 가 90 deg 에 가깝다 (뱃머리는 북, 가는 쪽은 동)
u = s(1);  v = s(2);  r = s(3);
x_n = s(4);  y_n = s(5);  psi = s(6);
U = sqrt(u*u + v*v);
beta = atan2(v, u);
c = psi + beta;
chi = atan2(sin(c), cos(c));
